simulink model "Foc"  (R2023b)
settings: Solver=FixedStepDiscrete  StartTime=0.0  StopTime=0.6  FixedStep=1e-6  MaxStep=1e-5  RelTol=1e-4
model workspace: external: MATLAB File D:\Simulink\Study\PMSM建模第三章\Foc_Params.m (data not in the file)
values from neighbouring files (symbols this model uses):
  B = 0.008    [CurrentHysteresis_Control_Params.m]    (also in Foc_Params.m; VF_Params.m)
  Ba = 0.013    [Foc_Params.m]
  flux = 0.175    [CurrentHysteresis_Control_Params.m]    (also in Foc_Params.m = 0.1827; VF_Params.m = 0.1827)
  fpwm = 10e3    (= 10000)    [Foc_Params.m]    (also in VF_Params.m)
  J = 0.0008    [CurrentHysteresis_Control_Params.m]    (also in Foc_Params.m = 0.003; VF_Params.m = 0.003)
  Kid = R*1100    (= 1053.8)    [Foc_Params.m]
  Kiq = R*1100    (= 1053.8)    [Foc_Params.m]
  Kiw = 0.14*50    (= 7)    [Foc_Params.m]
  Kpd = Ld*1100    (= 5.775)    [Foc_Params.m]
  Kpq = Lq*1100    (= 13.2)    [Foc_Params.m]
  Kpw = 0.14    [Foc_Params.m]
  Ld = 8.5e-3    (= 0.0085)    [CurrentHysteresis_Control_Params.m]    (also in Foc_Params.m = 0.00525; VF_Params.m = 0.00525)
  Lq = 8.5e-3    (= 0.0085)    [CurrentHysteresis_Control_Params.m]    (also in Foc_Params.m = 0.012; VF_Params.m = 0.012)
  Pn = 4    [CurrentHysteresis_Control_Params.m]    (also in Foc_Params.m; VF_Params.m)
  R = 2.875    [CurrentHysteresis_Control_Params.m]    (also in Foc_Params.m = 0.958; VF_Params.m = 0.958)
  Ts = 1e-5    (= 1e-05)    [Foc_Params.m]    (also in VF_Params.m)
  Vdc = 311    [Foc_Params.m]    (also in VF_Params.m)
undefined symbols (not defined in the file or in its folder): DiscIntNeverNeededParam
libraries: spsDCVoltageSourceLib x1, spsPermanentMagnetSynchronousMachineLib x1, simulink x1, spsUniversalBridgeLib x1, sps_lib x1
settings Model: Creator=123  LastModifiedBy=123

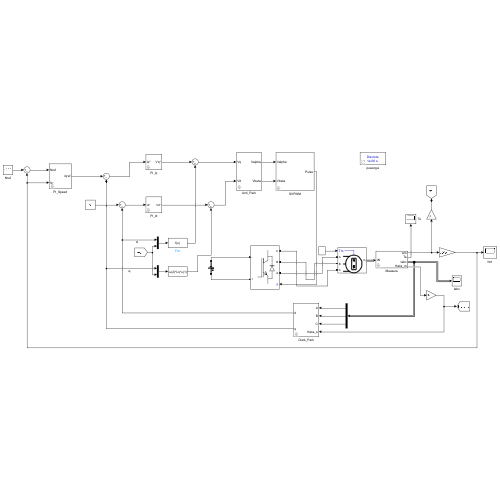
[thumbnail: Simulink's stored preview of the top-level diagram]
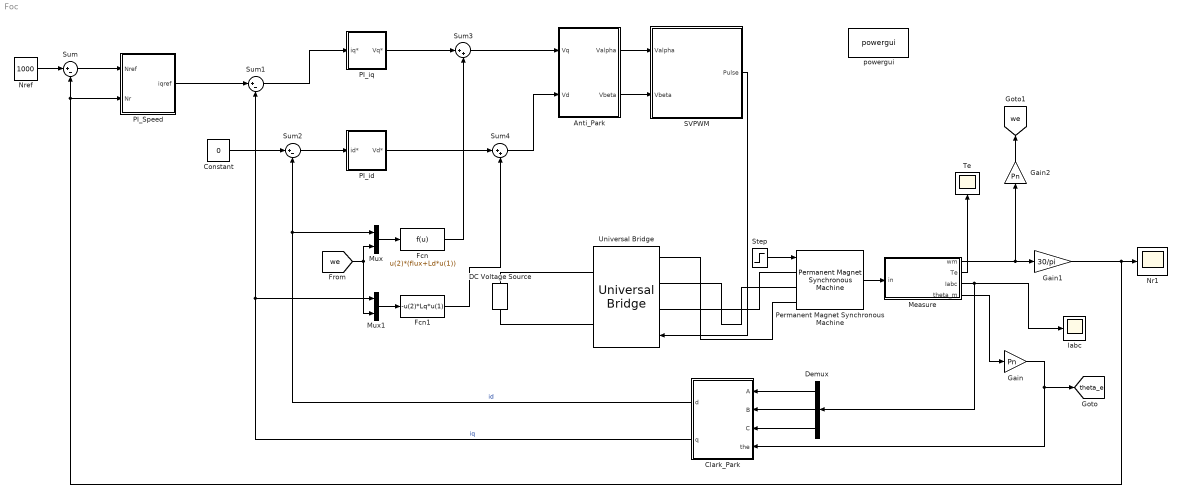
== system Foc ==
  Anti_Park : Subsystem
      mask DialogControl ParameterGroupVar Prompt: 参数
      mask Display:
      | port_label('input', 1, 'Vq');
      | port_label('input', 2, 'Vd');
      | port_label('output', 1, 'Valpha');
      | port_label('output', 2, 'Vbeta');
  Clark_Park : Subsystem
      mask DialogControl ParameterGroupVar Prompt: 参数
      mask Display:
      | port_label('input', 1, 'A');
      | port_label('input', 2, 'B');
      | port_label('input', 3, 'C');
      | port_label('input', 4, 'theta_e');
      | port_label('output', 1, 'd');
      | port_label('output', 2, 'q');
  Constant : Constant  Value=0
  DC Voltage Source : spsDCVoltageSourceLib/DC Voltage Source  Amplitude=Vdc  Measurements=None
  Demux : Demux  Outputs=3
  Fcn : Fcn  Expr=u(2)*(flux+Ld*u(1))
  Fcn1 : Fcn  Expr=-u(2)*Lq*u(1)
  Gain : Gain  Gain=Pn
  Gain1 : Gain  Gain=30/pi
  Gain2 : Gain  Gain=Pn
  Iabc : Scope
  Measure : Subsystem
      mask DialogControl ParameterGroupVar Prompt: 参数
      mask Display:
      | port_label('input', 1, 'IN');
      | port_label('output', 1, 'wm');
      | port_label('output', 2, 'Te');
      | port_label('output', 3, 'Iabc');
      | port_label('output', 4, 'theta_m');
  Mux : Mux  Inputs=2
  Mux1 : Mux  Inputs=2
  Nr1 : Scope
  Nref : Constant  Value=1000
  PI_Speed : Subsystem  mask{Kpw=Kpw, Kiw=Kiw, Up=30, Low=-30, Ts=Ts}
      mask prompts: Up "上限"; Low "下限"; Ts "采样时间"
      mask DialogControl ParameterGroupVar Prompt: 参数
      mask Display:
      | port_label('input', 2, 'Nr');
      | port_label('input', 1, 'Nref');
      | port_label('output', 1, 'iqref');
  PI_id : Subsystem  mask{Kpd=Kpd, Kid=Kid, Up=311*0.9*sqrt(1/3), Low=-311*0.9*sqrt(1/3), Ts=Ts}
      mask prompts: Up "上限"; Low "下限"; Ts "采样时间"
      mask DialogControl ParameterGroupVar Prompt: 参数
  PI_iq : Subsystem  mask{Kpq=Kpq, Kiq=Kiq, Up=311*0.9*sqrt(1/3), Low=-311*0.9*sqrt(1/3), Ts=Ts}
      mask prompts: Up "上限"; Low "下限"; Ts "采样时间"
      mask DialogControl ParameterGroupVar Prompt: 参数
      mask Display:
      | port_label('input', 1, 'iq*');
      | port_label('output', 1, 'Vq*');
  Permanent Magnet Synchronous Machine : spsPermanentMagnetSynchronousMachineLib/Permanent Magnet Synchronous Machine  NbPhases=3  FluxDistribution=Sinusoidal  RotorType=Salient-pole  MechanicalLoad=Torque Tm  PresetModel=No  ShowDetailedParameters=on  MeasurementBus=off  Resistance=R  Inductance=8.5e-3  dqInductances=[Ld,Lq]  La=0.000395  MachineConstant=Flux linkage established by magnets (V.s)  Flux=flux  VoltageCst=132.5525  TorqueCst=1.0962  Flat=120  Mechanical=[J B Pn 0]  PolePairs=4  InitialConditions=[0,0, 0,0]  InitialConditions5ph=[0 0 0 0 0 0]  RefAngle=Aligned with phase A axis (original Park)  IterativeDiscreteModel=Trapezoidal robust  TsBlock=-1  TsPowergui=0
  SVPWM : Subsystem  mask(SVPWM){udc_ref=Vdc, tpwm_ref=1/fpwm}
      mask prompts: udc_ref "DC bus voltage (V)"; tpwm_ref "PWM period (s)"
      mask help: Amplitude-invariant alpha/beta voltage references in volts. Pulse order: A upper, A lower, B upper, B lower, C upper, C lower. Ideal complementary gates; no dead time.
      mask Display: port_label('input',1,'Valpha');port_label('input',2,'Vbeta');port_label('output',1,'Pulse');
  Step : Step  Time=0.2  After=10  SampleTime=0
  Sum : Sum  Inputs=|+-
  Sum1 : Sum  Inputs=|+-
  Sum2 : Sum  Inputs=|+-
  Sum3 : Sum  Inputs=|++
  Sum4 : Sum  Inputs=|++
  Te : Scope
  Universal Bridge : spsUniversalBridgeLib/Universal Bridge  Arms=3  SnubberResistance=1e5  SnubberCapacitance=inf  Device=IGBT / Diodes  Ron=1e-3  Lon=0  ForwardVoltages="[  0  0  ]"  ForwardVoltage=0  GTOparameters=[ 10e-6 , 20e-6 ]  IGBTparameters=[ 1e-6 , 2e-6 ]  Measurements=None  Measurements_2=None  converterType=Rectifier
  powergui : sps_lib/powergui  Priority=1  SimulationMode=Discrete  SampleTime=1e-6  frequency=60  Iterations=50  frequencyindice=0  Pbase=100e6  ErrMax=1e-4  UnitsV=kV  UnitsW=MW  buscounter=0  FunctionMessages=off  echomessages=off  EnableUseOfTLC=off  CurrentSourceSwitches=off  DisableSnubberDevices=off  DisableRonSwitches=off  DisableVfSwitches=off  DisplayEquations=off  AutomaticDiscreteSolvers=off  SolverType=Tustin/Backward Euler (TBE)  Interpol=off  ExternalGateDelay=off  methode=off  Ts=100  x0status=blocks  SPID=on  SwTol=0  HookPort=off  NonlinearTolerance=1e-4  nMaxIteration=100  ContinueOnMaxIteration=off  RestoreLinks=warning  ResistiveCurrentMeasurement=off  Frange=[0:2:500]  Ylog=off  Xlog=on  ShowGrid=off  save=off  variable=ZData  structure=0  ZoomFFT=off  StartTime=0.0  cycles=1  DisplayStyle=1  fundamental=60  FreqAxis=off  MaxFrequency=1000  frequencyindicesteady=1  RmsSteady=1  display=off
  tag scope: theta_e=global, we=global
  wires:
  Step/1 -> Permanent Magnet Synchronous Machine/1
  SVPWM/1(Pulse) -> Universal Bridge/1
  Measure/1(wm) -> Gain1/1, Gain2/1
  Gain1/1 -> Nr1/1, PI_Speed/2(Nr), Sum/2
  Measure/4(theta_m) -> Gain/1
  Measure/3(Iabc) -> Demux/1, Iabc/1
  Permanent Magnet Synchronous Machine/1 -> Measure/1(in)
  Measure/2(Te) -> Te/1
  Anti_Park/1(Valpha) -> SVPWM/1(Valpha)
  Anti_Park/2(Vbeta) -> SVPWM/2(Vbeta)
  Gain/1 -> Clark_Park/4(the), [theta_e]
  Nref/1 -> Sum/1
  PI_Speed/1(iqref) -> Sum1/1
  Constant/1 -> Sum2/1
  Sum1/1 -> PI_iq/1(iq*)
  Sum2/1 -> PI_id/1(id*)
  PI_iq/1(Vq*) -> Sum3/1
  PI_id/1(Vd*) -> Sum4/1
  Gain2/1 -> [we]
  [we] -> Mux1/2, Mux/2
  Mux/1 -> Fcn/1
  Fcn/1 -> Sum3/2
  Mux1/1 -> Fcn1/1
  Fcn1/1 -> Sum4/2
  Sum4/1 -> Anti_Park/2(Vd)
  Sum3/1 -> Anti_Park/1(Vq)
  Sum/1 -> PI_Speed/1(Nref)
  Demux/1 -> Clark_Park/1(A)
  Demux/2 -> Clark_Park/2(B)
  Demux/3 -> Clark_Park/3(C)
  Clark_Park/1(d) -> Mux/1, Sum2/2  "id"
  Clark_Park/2(q) -> Mux1/1, Sum1/2  "iq"
  connections:
  DC Voltage Source/RConn1 -- Universal Bridge/RConn1
  Universal Bridge/LConn1 -- Permanent Magnet Synchronous Machine/LConn1
  DC Voltage Source/LConn1 -- Universal Bridge/RConn2
  Universal Bridge/LConn3 -- Permanent Magnet Synchronous Machine/LConn3
  Universal Bridge/LConn2 -- Permanent Magnet Synchronous Machine/LConn2

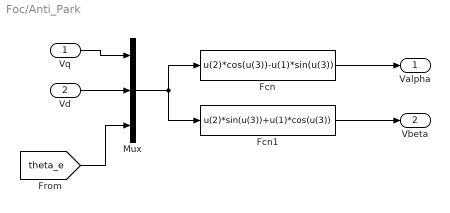
== system Foc/Anti_Park ==
  Vq : Inport
  Vd : Inport  Port=2
  Fcn : Fcn  Expr=u(2)*cos(u(3))-u(1)*sin(u(3))
  Fcn1 : Fcn  Expr=u(2)*sin(u(3))+u(1)*cos(u(3))
  Mux : Mux  Inputs=3
  Valpha : Outport
  Vbeta : Outport  Port=2
  wires:
  Vq/1 -> Mux/1
  Vd/1 -> Mux/2
  Mux/1 -> Fcn1/1, Fcn/1
  Fcn/1 -> Valpha/1
  Fcn1/1 -> Vbeta/1
  [theta_e] -> Mux/3

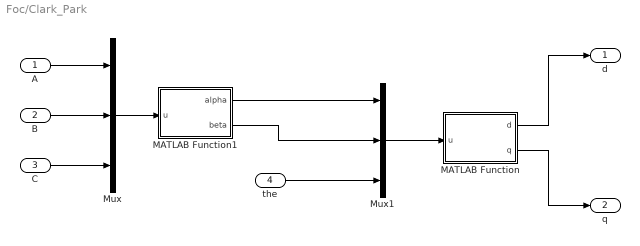
== system Foc/Clark_Park ==
  A : Inport
  B : Inport  Port=2
  C : Inport  Port=3
  the : Inport  Port=4
  MATLAB Function : MATLAB Function  TreatAsAtomicUnit=on
  MATLAB Function1 : MATLAB Function  TreatAsAtomicUnit=on
  Mux : Mux  Inputs=3
  Mux1 : Mux  Inputs=3
  d : Outport
  q : Outport  Port=2
  wires:
  C/1 -> Mux/3
  Mux1/1 -> MATLAB Function/1(u)
  A/1 -> Mux/1
  the/1 -> Mux1/3
  B/1 -> Mux/2
  Mux/1 -> MATLAB Function1/1(u)
  MATLAB Function/2(q) -> q/1
  MATLAB Function1/2(beta) -> Mux1/2
  MATLAB Function/1(d) -> d/1
  MATLAB Function1/1(alpha) -> Mux1/1

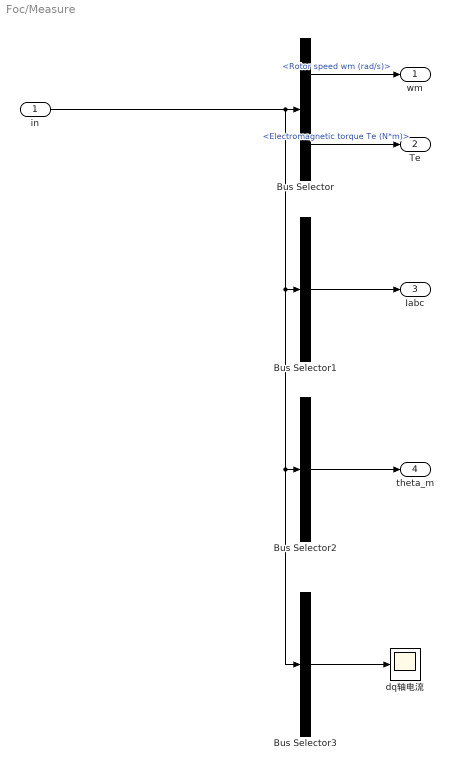
== system Foc/Measure ==
  in : Inport
  Bus Selector : BusSelector  OutputSignals=Rotor speed wm (rad/s),Electromagnetic torque Te (N*m)
  Bus Selector1 : BusSelector  OutputSignals=Stator current is_a (A),Stator current is_b (A),Stator current is_c (A)  OutputAsBus=on
  Bus Selector2 : BusSelector  OutputSignals=Rotor angle thetam (rad)  OutputAsBus=on
  Bus Selector3 : BusSelector  OutputSignals=Stator current is_d (A),Stator current is_q (A)  OutputAsBus=on
  dq轴电流 : Scope
  wm : Outport
  Te : Outport  Port=2
  Iabc : Outport  Port=3
  theta_m : Outport  Port=4
  wires:
  in/1 -> Bus Selector3/1, Bus Selector2/1, Bus Selector1/1, Bus Selector/1
  Bus Selector/1 -> wm/1  "<Rotor speed wm (rad/s)>"
  Bus Selector/2 -> Te/1  "<Electromagnetic torque Te (N*m)>"
  Bus Selector1/1 -> Iabc/1
  Bus Selector2/1 -> theta_m/1
  Bus Selector3/1 -> dq轴电流/1

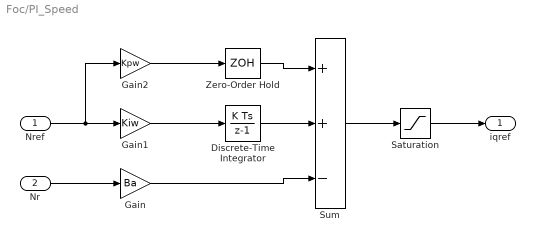
== system Foc/PI_Speed ==
  Nref : Inport
  Nr : Inport  Port=2
  Discrete-Time Integrator : DiscreteIntegrator  SampleTime=Ts  ICPrevOutput=DiscIntNeverNeededParam  ICPrevScaledInput=DiscIntNeverNeededParam
  Gain : Gain  Gain=Ba
  Gain1 : Gain  Gain=Kiw
  Gain2 : Gain  Gain=Kpw
  Saturation : Saturate  UpperLimit=Up  LowerLimit=Low
  Sum : Sum  Inputs=++-
  Zero-Order Hold : ZeroOrderHold  SampleTime=Ts
  iqref : Outport
  wires:
  Nr/1 -> Gain/1
  Nref/1 -> Gain1/1, Gain2/1
  Gain2/1 -> Zero-Order Hold/1
  Gain1/1 -> Discrete-Time Integrator/1
  Zero-Order Hold/1 -> Sum/1
  Discrete-Time Integrator/1 -> Sum/2
  Gain/1 -> Sum/3
  Sum/1 -> Saturation/1
  Saturation/1 -> iqref/1

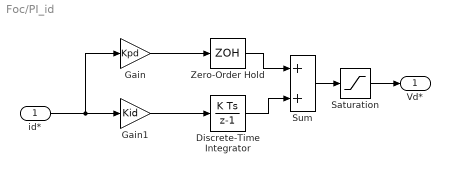
== system Foc/PI_id ==
  id* : Inport
  Discrete-Time Integrator : DiscreteIntegrator  SampleTime=Ts  ICPrevOutput=DiscIntNeverNeededParam  ICPrevScaledInput=DiscIntNeverNeededParam
  Gain : Gain  Gain=Kpd
  Gain1 : Gain  Gain=Kid
  Saturation : Saturate  UpperLimit=Up  LowerLimit=Low
  Sum : Sum
  Zero-Order Hold : ZeroOrderHold  SampleTime=Ts
  Vd* : Outport
  wires:
  Sum/1 -> Saturation/1
  Gain/1 -> Zero-Order Hold/1
  Zero-Order Hold/1 -> Sum/1
  Discrete-Time Integrator/1 -> Sum/2
  id*/1 -> Gain1/1, Gain/1
  Saturation/1 -> Vd*/1
  Gain1/1 -> Discrete-Time Integrator/1

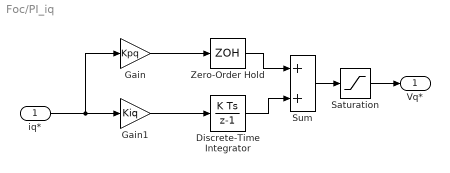
== system Foc/PI_iq ==
  iq* : Inport
  Discrete-Time Integrator : DiscreteIntegrator  SampleTime=Ts  ICPrevOutput=DiscIntNeverNeededParam  ICPrevScaledInput=DiscIntNeverNeededParam
  Gain : Gain  Gain=Kpq
  Gain1 : Gain  Gain=Kiq
  Saturation : Saturate  UpperLimit=Up  LowerLimit=Low
  Sum : Sum
  Zero-Order Hold : ZeroOrderHold  SampleTime=Ts
  Vq* : Outport
  wires:
  iq*/1 -> Gain1/1, Gain/1
  Gain/1 -> Zero-Order Hold/1
  Gain1/1 -> Discrete-Time Integrator/1
  Zero-Order Hold/1 -> Sum/1
  Discrete-Time Integrator/1 -> Sum/2
  Sum/1 -> Saturation/1
  Saturation/1 -> Vq*/1

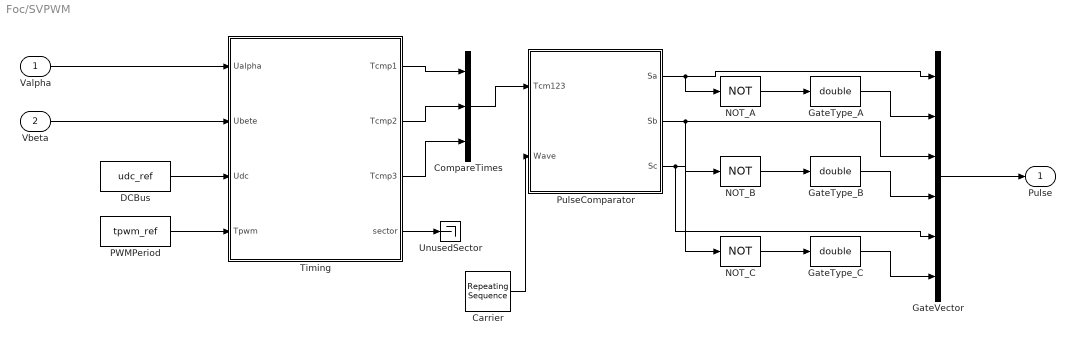
== system Foc/SVPWM ==
  Valpha : Inport
  Vbeta : Inport  Port=2
  Carrier : simulink/Sources/Repeating Sequence  rep_seq_t=[0 tpwm_ref/2 tpwm_ref]  rep_seq_y=[0 tpwm_ref/2 0]
  CompareTimes : Mux  Inputs=3
  DCBus : Constant  Value=udc_ref
  GateType_A : DataTypeConversion  OutDataTypeStr=double  SaturateOnIntegerOverflow=off  RndMeth=Floor
  GateType_B : DataTypeConversion  OutDataTypeStr=double  SaturateOnIntegerOverflow=off  RndMeth=Floor
  GateType_C : DataTypeConversion  OutDataTypeStr=double  SaturateOnIntegerOverflow=off  RndMeth=Floor
  GateVector : Mux  Inputs=6
  NOT_A : Logic  Operator=NOT  AllPortsSameDT=off  OutDataTypeStr=boolean
  NOT_B : Logic  Operator=NOT  AllPortsSameDT=off  OutDataTypeStr=boolean
  NOT_C : Logic  Operator=NOT  AllPortsSameDT=off  OutDataTypeStr=boolean
  PWMPeriod : Constant  Value=tpwm_ref
  PulseComparator : Subsystem
  Timing : MATLAB Function  TreatAsAtomicUnit=on
  UnusedSector : Terminator
  Pulse : Outport
  wires:
  Valpha/1 -> Timing/1(Ualpha)
  Vbeta/1 -> Timing/2(Ubete)
  DCBus/1 -> Timing/3(Udc)
  PWMPeriod/1 -> Timing/4(Tpwm)
  Timing/1(Tcmp1) -> CompareTimes/1
  Timing/2(Tcmp2) -> CompareTimes/2
  Timing/3(Tcmp3) -> CompareTimes/3
  Timing/4(sector) -> UnusedSector/1
  CompareTimes/1 -> PulseComparator/1(Tcm123)
  Carrier/1 -> PulseComparator/2(Wave)
  PulseComparator/1(Sa) -> GateVector/1, NOT_A/1
  NOT_A/1 -> GateType_A/1
  GateType_A/1 -> GateVector/2
  PulseComparator/2(Sb) -> GateVector/3, NOT_B/1
  NOT_B/1 -> GateType_B/1
  GateType_B/1 -> GateVector/4
  PulseComparator/3(Sc) -> GateVector/5, NOT_C/1
  NOT_C/1 -> GateType_C/1
  GateType_C/1 -> GateVector/6
  GateVector/1 -> Pulse/1

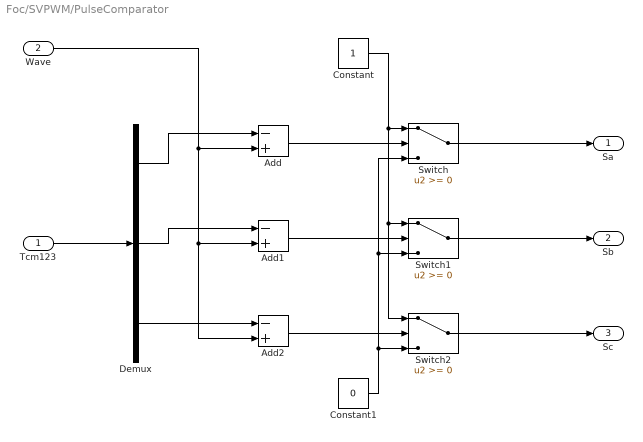
== system Foc/SVPWM/PulseComparator ==
  Tcm123 : Inport
  Wave : Inport  Port=2
  Add : Sum  Inputs=-+
  Add1 : Sum  Inputs=-+
  Add2 : Sum  Inputs=-+
  Constant : Constant
  Constant1 : Constant  Value=0
  Demux : Demux  Outputs=3
  Switch : Switch  SaturateOnIntegerOverflow=off  InputSameDT=off
  Switch1 : Switch  SaturateOnIntegerOverflow=off  InputSameDT=off
  Switch2 : Switch  SaturateOnIntegerOverflow=off  InputSameDT=off
  Sa : Outport
  Sb : Outport  Port=2
  Sc : Outport  Port=3
  wires:
  Switch2/1 -> Sc/1
  Switch1/1 -> Sb/1
  Switch/1 -> Sa/1
  Constant1/1 -> Switch/3, Switch1/3, Switch2/3
  Constant/1 -> Switch/1, Switch1/1, Switch2/1
  Add/1 -> Switch/2
  Add1/1 -> Switch1/2
  Add2/1 -> Switch2/2
  Demux/3 -> Add2/1
  Demux/2 -> Add1/1
  Demux/1 -> Add/1
  Wave/1 -> Add2/2, Add1/2, Add/2
  Tcm123/1 -> Demux/1

== matlab function Foc/Clark_Park/MATLAB Function1 ==
  data: u input; alpha output; beta output
function [alpha, beta] = fcn(u)

alpha = (u(1)-0.5*(u(2)+u(3)))*2/3;
beta  = sqrt(3)/2*(u(2)-u(3))*2/3;

end

== matlab function Foc/Clark_Park/MATLAB Function ==
  data: u input; d output; q output
function [d,q]  = fcn(u)

d = u(1)*cos(u(3))+u(2)*sin(u(3));
q = -u(1)*sin(u(3))+u(2)*cos(u(3));

end

== matlab function Foc/SVPWM/Timing ==
  data: Ualpha input; Tcmp1 output; Ubete input; Udc input; Tpwm input; Tcmp2 output; Tcmp3 output; sector output
function [Tcmp1,Tcmp2,Tcmp3,sector] = fcn(Ualpha,Ubete,Udc,Tpwm)

%变量初始化

Tcmp1 = 0;
Tcmp2 = 0;
Tcmp3 = 0;
sector = 0;
T1 = 0;
T2 = 0;

%扇区选择

Uref1 = Ubete;
Uref2 = (sqrt(3)*Ualpha - Ubete)/2;
Uref3 = (-sqrt(3)*Ualpha - Ubete)/2;

if(Uref1 > 0)
    sector = 1;
end
if(Uref2 > 0)
    sector = sector + 2;
end
if(Uref3 > 0)
    sector = sector + 4;
end

%非零矢量和零矢量作用时间

X = sqrt(3)*Ubete*Tpwm/Udc;
Y = Tpwm/Udc*(3/2*Ualpha + sqrt(3)/2*Ubete);
Z = Tpwm/Udc*(-3/2*Ualpha + sqrt(3)/2*Ubete);

switch(sector)
    case 1
        T1 = Z;T2 = Y;
    case 2
        T1 = Y;T2 = -X;
    case 3
        T1 = -Z;T2 = X;
    case 4
        T1 = -X;T2 = Z;
    case 5
        T1 = X;T2 = -Y;
    case 6
        T1 = -Y;T2 = -Z;
end

%过调制处理，变成占空比处理

if (T1+T2>Tpwm)
    scale = Tpwm/(T1+T2);
    T1 = T1*scale;
    T2 = T2*scale;
else
    T1 = T1;
    T2 = T2;
end

%扇区矢量切换点确定

ta = (Tpwm-(T1+T2))/4.0;
tb = ta+T1/2;
tc = tb+T2/2;

switch(sector)
    case 1
        Tcmp1 = tb;
        Tcmp2 = ta;
        Tcmp3 = tc;
    case 2
        Tcmp1 = ta;
        Tcmp2 = tc;
        Tcmp3 = tb;
    case 3
        Tcmp1 = ta;
        Tcmp2 = tb;
        Tcmp3 = tc;
    case 4
        Tcmp1 = tc;
        Tcmp2 = tb;
        Tcmp3 = ta;
    case 5
        Tcmp1 = tc;
        Tcmp2 = ta;
        Tcmp3 = tb;
    case 6
        Tcmp1 = tb;
        Tcmp2 = tc;
        Tcmp3 = ta;
end
end
